simulink model "PID_temp"  (R2025b)
settings: Solver=VariableStepAuto  StartTime=0.0  StopTime=10.0  RelTol=1e-3
libraries: simulink x1
settings Model: Creator=alosw  LastModifiedBy=alosw

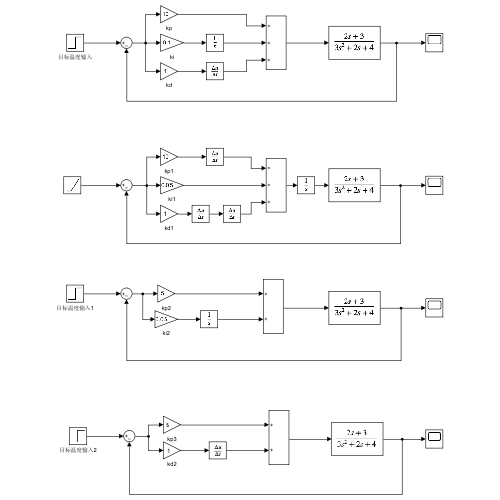
[thumbnail: Simulink's stored preview of the top-level diagram]
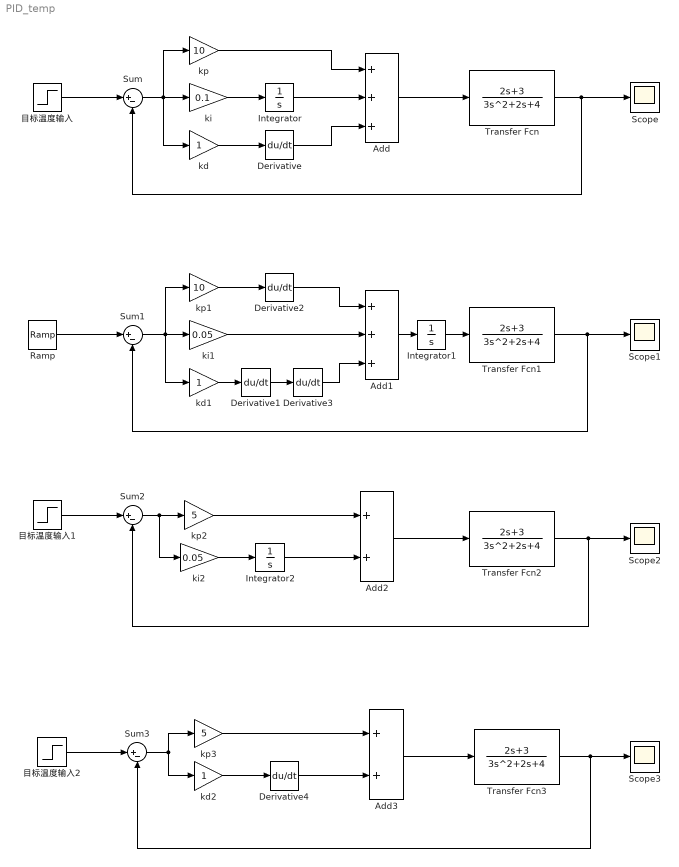
== system PID_temp ==
  Add : Sum  Inputs=+++
  Add1 : Sum  Inputs=+++
  Add2 : Sum
  Add3 : Sum
  Derivative{,1..4} (5 alike) : Derivative
  Integrator : Integrator
  Integrator1 : Integrator
  Integrator2 : Integrator
  Ramp : simulink/Sources/Ramp  slope=1  start=0  InitialOutput=0
  Scope{,1..3} (4 alike) : Scope
      Scope settings: ActiveDisplayYMinimum=5.7521460987720108  ActiveDisplayYMaximum=12.043294758388637
      Scope1 settings: ActiveDisplayYMinimum=17.641697016875305  ActiveDisplayYMaximum=19.366269744288942
      Scope2 settings: ActiveDisplayYMinimum=-2.3895185190311965  ActiveDisplayYMaximum=12.120892804767063  DataLoggingVariableName=ScopeData2
      Scope3 settings: ActiveDisplayYMinimum=-1.5601667950463209  ActiveDisplayYMaximum=10.173547115199225  DataLoggingVariableName=ScopeData3
  Sum{,1..3} (4 alike) : Sum  Inputs=|+-
  Transfer Fcn{,1..3} (4 alike) : TransferFcn  Numerator=[2 3]  Denominator=[3 2 4]
  kd : Gain
  kd1 : Gain
  kd2 : Gain
  ki : Gain  Gain=0.1
  ki1 : Gain  Gain=0.05
  ki2 : Gain  Gain=0.05
  kp : Gain  Gain=10
  kp1 : Gain  Gain=10
  kp2 : Gain  Gain=5
  kp3 : Gain  Gain=5
  目标温度输入 : Step  Time=0.1  After=10  SampleTime=0
  目标温度输入1 : Step  Time=0.1  After=10  SampleTime=0
  目标温度输入2 : Step  Time=0.1  After=10  SampleTime=0
  wires:
  目标温度输入/1 -> Sum/1
  ki/1 -> Integrator/1
  kd/1 -> Derivative/1
  Sum/1 -> kd/1, ki/1, kp/1
  Derivative/1 -> Add/3
  Integrator/1 -> Add/2
  kp/1 -> Add/1
  Add/1 -> Transfer Fcn/1
  Transfer Fcn/1 -> Sum/2, Scope/1
  kd1/1 -> Derivative1/1
  Ramp/1 -> Sum1/1
  ki1/1 -> Add1/2
  Sum1/1 -> kd1/1, ki1/1, kp1/1
  Transfer Fcn1/1 -> Sum1/2, Scope1/1
  kp1/1 -> Derivative2/1
  Derivative2/1 -> Add1/1
  Derivative1/1 -> Derivative3/1
  Derivative3/1 -> Add1/3
  Integrator1/1 -> Transfer Fcn1/1
  Add1/1 -> Integrator1/1
  Add2/1 -> Transfer Fcn2/1
  目标温度输入1/1 -> Sum2/1
  Integrator2/1 -> Add2/2
  kp2/1 -> Add2/1
  ki2/1 -> Integrator2/1
  Sum2/1 -> ki2/1, kp2/1
  Transfer Fcn2/1 -> Sum2/2, Scope2/1
  Add3/1 -> Transfer Fcn3/1
  kd2/1 -> Derivative4/1
  目标温度输入2/1 -> Sum3/1
  kp3/1 -> Add3/1
  Derivative4/1 -> Add3/2
  Sum3/1 -> kd2/1, kp3/1
  Transfer Fcn3/1 -> Scope3/1, Sum3/2
